simulink model "HW1_C"  (R2023b)
settings: Solver=VariableStepAuto  StartTime=0.0  StopTime=1000  RelTol=1e-3
libraries: commdigbbndam3 x3, commchan3 x2, commsink2 x2, dspxfrm3 x2, commrandsrc3 x1
settings Model: Creator=chang  LastModifiedBy=chang
settings SFSimCC: SimCustomHeaderCode="#include \"srfft_head.h\""
settings SFSimCC: SimUserSources=|
  | srfft.c
  | bit_reverse.c
  | log2_int.c
  | twiddle_factor.c
  | complex_mul.c

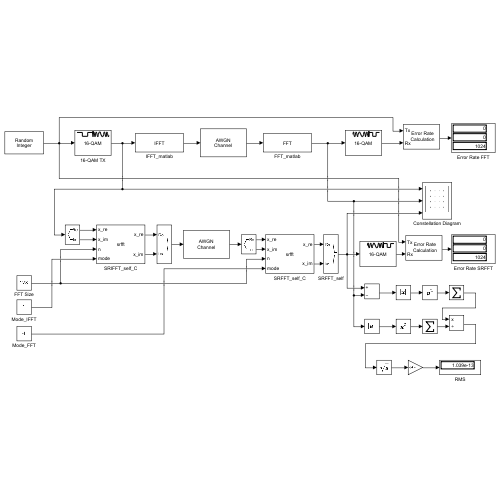
[thumbnail: Simulink's stored preview of the top-level diagram]
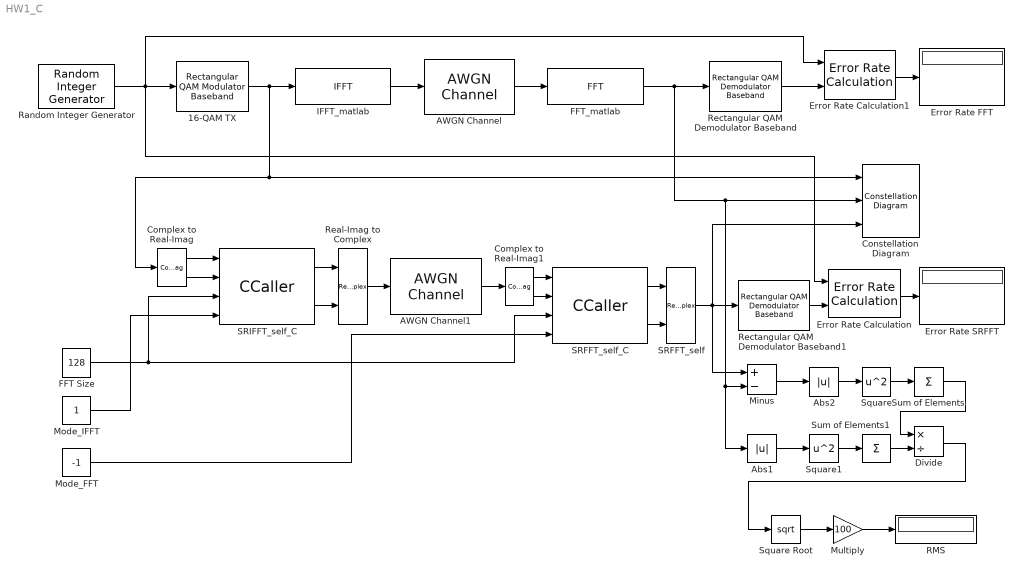
== system HW1_C ==
  16-QAM TX : commdigbbndam3/Rectangular QAM Modulator Baseband  M=16  InType=Integer  Enc=Gray  Mapping=[0:15]  PowType=Average Power  MinDist=2  AvgPow=1  PeakPow=1  Ph=0  outDtype=double  outWordLen=16  outUDDataType=sfix(16)  outFracLenMode=Best precision  outFracLen=15  outDataTypeStr=double  outLastDataTypeStr=double
  AWGN Channel : commchan3/AWGN Channel  LegacyMode=on  NoiseMethod="Signal to noise ratio  (SNR)"  noiseMode="Signal to noise ratio  (Eb/No)"  EbNo=40  EsNo=10  SNR=10  BitsPerSymbol=2  SignalPower=1  SamplesPerSymbol=1  SymbolPeriod=1  VarianceSource=Parameter  Variance=1  RandomStream=Global stream  Seed=67  SimulateUsing=Code generation
  AWGN Channel1 : commchan3/AWGN Channel  LegacyMode=on  NoiseMethod="Signal to noise ratio  (SNR)"  noiseMode="Signal to noise ratio  (Eb/No)"  EbNo=40  EsNo=10  SNR=10  BitsPerSymbol=2  SignalPower=1  SamplesPerSymbol=1  SymbolPeriod=1  VarianceSource=Parameter  Variance=1  RandomStream=Global stream  Seed=67  SimulateUsing=Code generation
  Abs1 : Abs  SaturateOnIntegerOverflow=off
  Abs2 : Abs  SaturateOnIntegerOverflow=off
  Complex to Real-Imag : ComplexToRealImag
  Complex to Real-Imag1 : ComplexToRealImag
  Constellation Diagram : ConstellationDiagram  NumInputPorts=3  WindowPosition=[1504.000000,416.000000,600.000000,600.000000,]  ScopeFrameLocation=window  ReferenceConstellation="{[0.7071+0.7071i          -0.7071+0.7071i          -0.7071-0.7071i            0.707-0.7071i][0.7071+0.7071i          -0.7071+0.7071i          -0.7071-0.7071i            0.707-0.7071i][0.7071+0.7071i          -0.7071+0.7071i          -0.7071-0.7071i            0.707-0.7071i]}"  ShowLegend=on
  Divide : Product  Inputs=*/
  Error Rate Calculation : commsink2/Error Rate Calculation  N=0  st_delay=0  cp_mode=Entire frame  subframe=[]  PMode=Port  WsName=ErrorVec  RsMode2=off  stop=off  numErr=100  maxBits=1e6
      settings: LibrarySourceBlock=|
      | commhdlsink/Error Rate
      | Calculation
  Error Rate Calculation1 : commsink2/Error Rate Calculation  N=0  st_delay=0  cp_mode=Entire frame  subframe=[]  PMode=Port  WsName=ErrorVec  RsMode2=off  stop=off  numErr=100  maxBits=1e6
      settings: LibrarySourceBlock=|
      | commhdlsink/Error Rate
      | Calculation
  Error Rate FFT : Display
  Error Rate SRFFT : Display
  FFT Size : Constant  Value=128
  FFT_matlab : dspxfrm3/FFT  FFTImplementation=Auto  CompMethod=Table lookup  TableOpt=NEW  TableOptActive=Speed  BitRevOrder=off  Normalize=off  InheritFFTLength=on  FFTLength=64  WrapInput=on  roundingMode=Floor  overflowMode=off  firstCoeffDataTypeStr=Inherit: Same word length as input  firstCoeffLastDataTypeStr=Inherit: Same word length as input  outputMin=[]  outputMax=[]
  IFFT_matlab : dspxfrm3/IFFT  FFTImplementation=Auto  CompMethod=Table lookup  TableOpt=NEW  TableOptActive=Speed  BitRevOrder=off  cs_in=off  Normalize=on  InheritFFTLength=on  FFTLength=64  WrapInput=on  mode=Complex  outSamplingMode=Sample based  roundingMode=Floor  overflowMode=off  firstCoeffDataTypeStr=Inherit: Same word length as input  firstCoeffLastDataTypeStr=Inherit: Same word length as input  outputMin=[]  outputMax=[]
  Minus : Sum  Inputs=+-
  Mode_FFT : Constant  Value=-1
  Mode_IFFT : Constant
  Multiply : Gain  Gain=100
  RMS : Display
  Random Integer Generator : commrandsrc3/Random Integer Generator  SetSize=16  SeedSource=Parameter  Seed=36  SampleTime=1  SamplesPerFrame=128  OutputDataType=double  SimulateUsing=Interpreted execution
  Real-Imag to Complex : RealImagToComplex
  Rectangular QAM Demodulator Baseband : commdigbbndam3/Rectangular QAM Demodulator Baseband  M=16  OutType=Integer  DecType=Hard decision  VarSource=Dialog  Variance=1  Dec=Gray  Mapping=[0:15]  PowType=Average Power  MinDist=2  AvgPow=1  PeakPow=1  Ph=0  outDtype1=Inherit via internal rule  outDtype2=Inherit via internal rule  derotateFactorWordLen=16  derotateFactorDataTypeStr=Inherit: Same word length as input  derotateFactorLastDataTypeStr=Inherit: Same word length as input  denormFactorWordLen=16  denormFactorDataTypeStr=Inherit: Same word length as input  denormFactorLastDataTypeStr=Inherit: Same word length as input  prodOutWordLen=32  prodOutOverflowMode=Wrap  prodOutRoundingMode=Floor  prodOutOvFlMode=off  prodOutOvFlModeLastStrValue=off  sumWordLen=32
  Rectangular QAM Demodulator Baseband1 : commdigbbndam3/Rectangular QAM Demodulator Baseband  M=16  OutType=Integer  DecType=Hard decision  VarSource=Dialog  Variance=1  Dec=Gray  Mapping=[0:15]  PowType=Average Power  MinDist=2  AvgPow=1  PeakPow=1  Ph=0  outDtype1=Inherit via internal rule  outDtype2=Inherit via internal rule  derotateFactorWordLen=16  derotateFactorDataTypeStr=Inherit: Same word length as input  derotateFactorLastDataTypeStr=Inherit: Same word length as input  denormFactorWordLen=16  denormFactorDataTypeStr=Inherit: Same word length as input  denormFactorLastDataTypeStr=Inherit: Same word length as input  prodOutWordLen=32  prodOutOverflowMode=Wrap  prodOutRoundingMode=Floor  prodOutOvFlMode=off  prodOutOvFlModeLastStrValue=off  sumWordLen=32
  SRFFT_self : RealImagToComplex
  SRFFT_self_C : CCaller  FunctionName=srfft  PortSpecificationStruct="%)30     .    : 4   8    (     @         %    \"     ,    !     0         %  0 \"0    $    _    07)G3F%M90  4&]R=$YA;64 4V-O<&4     26YD97@     5'EP90      4VEZ90      27-';&]B86P   X    P    !@    @    $          4    (     0    $    !         !   0!X    #@   #     &    \"     0         !0    @    !     0    $         $  ! '@    .    0     8    (    !          %    \"     $    +     0         0    \"P   $EN<'5T3W5T<'5T       .    .     8    (    !@         %    \"     $    !     0         )    \"               #@   $     &    \"     0         !0    @    !    #     $         $     P   !\"=7,Z($-O;7!L97@     #@   #     &    \"     0         !0    @    !     @    $         $  \" \"TQ   .    ,     8    (    \"0(        %    \"     $    !     0         \"  $       X    P    !@    @    $          4    (     0    $    !         !   0!N    #@   #     &    \"     0         !0    @    !     0    $         $  ! &X    .    .     8    (    !          %    \"     $    %     0         0    !0   $EN<'5T    #@   #@    &    \"     8         !0    @    !     0    $         \"0    @           #P/PX    X    !@    @    $          4    (     0    8    !         !     &    9&]U8FQE   .    ,     8    (    !          %    \"     $    !     0         0  $ ,0    X    P    !@    @    ) @        4    (     0    $    !          (  0      #@   #     &    \"     0         !0    @    !    !     $         $  $ &UO9&4.    ,     8    (    !          %    \"     $    $     0         0  0 ;6]D90X    X    !@    @    $          4    (     0    4    !         !     %    26YP=70    .    .     8    (    !@         %    \"     $    !     0         )    \"             ! #@   #@    &    \"     0         !0    @    !    !@    $         $     8   !D;W5B;&4   X    P    !@    @    $          4    (     0    $    !         !   0 Q    #@   #     &    \"     D\"        !0    @    !     0    $          @ !"
  SRIFFT_self_C : CCaller  FunctionName=srfft  PortSpecificationStruct="%)30     .    \" <   8    (     @         %    \"     0    !     0         %  0 \"0    $    _    07)G3F%M90  4&]R=$YA;64 4V-O<&4     26YD97@     5'EP90      4VEZ90      27-';&]B86P   X    P    !@    @    $          4    (     0    0    !         !  ! !X7W)E#@   #     &    \"     0         !0    @    !    !     $         $  $ 'A?<F4.    0     8    (    !          %    \"     $    +     0         0  ...(+2046 chars)"
  Square : Math  Operator=square
  Square Root : Sqrt
  Square1 : Math  Operator=square
  Sum of Elements : Sum  Inputs=+
  Sum of Elements1 : Sum  Inputs=+
  wires:
  IFFT_matlab/1 -> AWGN Channel/1
  AWGN Channel/1 -> FFT_matlab/1
  FFT_matlab/1 -> Rectangular QAM Demodulator Baseband/1, Minus/2, Abs1/1, Constellation Diagram/2
  16-QAM TX/1 -> IFFT_matlab/1, Complex to Real-Imag/1, Constellation Diagram/1
  AWGN Channel1/1 -> Complex to Real-Imag1/1
  SRIFFT_self_C/1 -> Real-Imag to Complex/1
  SRIFFT_self_C/2 -> Real-Imag to Complex/2
  Real-Imag to Complex/1 -> AWGN Channel1/1
  Mode_IFFT/1 -> SRIFFT_self_C/4
  FFT Size/1 -> SRIFFT_self_C/3, SRFFT_self_C/3
  Complex to Real-Imag/2 -> SRIFFT_self_C/2
  Complex to Real-Imag/1 -> SRIFFT_self_C/1
  Complex to Real-Imag1/1 -> SRFFT_self_C/1
  Complex to Real-Imag1/2 -> SRFFT_self_C/2
  Mode_FFT/1 -> SRFFT_self_C/4
  SRFFT_self_C/1 -> SRFFT_self/1
  SRFFT_self_C/2 -> SRFFT_self/2
  SRFFT_self/1 -> Rectangular QAM Demodulator Baseband1/1, Minus/1, Constellation Diagram/3
  Error Rate Calculation/1 -> Error Rate SRFFT/1
  Rectangular QAM Demodulator Baseband1/1 -> Error Rate Calculation/2
  Random Integer Generator/1 -> Error Rate Calculation1/1, Error Rate Calculation/1, 16-QAM TX/1
  Rectangular QAM Demodulator Baseband/1 -> Error Rate Calculation1/2
  Error Rate Calculation1/1 -> Error Rate FFT/1
  Minus/1 -> Abs2/1
  Abs2/1 -> Square/1
  Square/1 -> Sum of Elements/1
  Abs1/1 -> Square1/1
  Square1/1 -> Sum of Elements1/1
  Sum of Elements/1 -> Divide/1
  Sum of Elements1/1 -> Divide/2
  Divide/1 -> Square Root/1
  Square Root/1 -> Multiply/1
  Multiply/1 -> RMS/1
